simulink model "eml_hdl_design_patterns"  (R2026a)
settings: Solver=FixedStepDiscrete  StopTime=10
InitFcn:
  | errMsg  = ['\n\nThis model is only for demonstration purposes.\n\nPlease do not Simulate or code generate directly from this model. \n\nBefore generating code from this model please do copy the relevant blocks of interest from this model to a new model, place them in a subsystem, build a valid test bench around them.\n\nPlease refer to the example model ''eml_hdl_incrementer'' or HDLCoder documentation'];
  | error(sprintf(errMsg));
undefined symbols (not defined in the file or in its folder): C, gain_val, init_val, lower_limit, maxWordLength, thresh, upper_limit
libraries: simulink x2
(part 5 of 5)

== matlab function eml_hdl_design_patterns/Decoders/hierarchical_viterbi/PMU1/ACS ==
  settings: fimath=|
      | fimath(...
      |     'RoundMode', 'floor',...
      |     'OverflowMode', 'saturate',...
      |     'ProductMode', 'FullPrecision', 'ProductWordLength', 32,...
      |     'SumMode', 'FullPrecision', 'SumWordLength', 32,...
      |     'CastBeforeSum', true);
  data: nsm output; bm input; dec output; sm_reg input size=[1 64]
function [nsm,dec]  = ACSU(bm, sm_reg)
%--------------------------------------------------------------------------
%  ACS (Add-Compare-Select) block
%--------------------------------------------------------------------------

[nsm, dec] = acsunitbutterfly(bm, sm_reg);
   
end

%--------------------------------------------------------------------------
% ACS Unit Group(Add-Compare-Select)
% For each state in the trellis diagram, for each node in this state:
% 1. Add the branch metric to the paths merged to this node. 
% 2. Compare all the paths merged to this road
% 3. Select the path with the minimum path metric
%
% The following code is generated by a script 'generateviterbi.m'
% that generates trellis diagram for convolution code (7,171,133)
%--------------------------------------------------------------------------
function [nsm, dec] = acsunitbutterfly(bm, sm)

nsm = getfi(zeros(1,64),1, 12, 6);
dec = getfi(zeros(1,64),0, 1,  0);

%----------------------------------------------------
% 000000   -> 00 -> 000000   000001   -> 11 -> 000000   
%----------------------------------------------------
[nsm(1), dec(1)] = acsunit(bm(1),bm(4),sm(1),sm(2));
%----------------------------------------------------
% 000000   -> 11 -> 100000   000001   -> 00 -> 100000   
%----------------------------------------------------
[nsm(33), dec(33)] = acsunit(bm(4),bm(1),sm(1),sm(2));
%----------------------------------------------------
% 000010   -> 01 -> 000001   000011   -> 10 -> 000001   
%----------------------------------------------------
[nsm(2), dec(2)] = acsunit(bm(2),bm(3),sm(3),sm(4));
%----------------------------------------------------
% 000010   -> 10 -> 100001   000011   -> 01 -> 100001   
%----------------------------------------------------
[nsm(34), dec(34)] = acsunit(bm(3),bm(2),sm(3),sm(4));
%----------------------------------------------------
% 000100   -> 00 -> 000010   000101   -> 11 -> 000010   
%----------------------------------------------------
[nsm(3), dec(3)] = acsunit(bm(1),bm(4),sm(5),sm(6));
%----------------------------------------------------
% 000100   -> 11 -> 100010   000101   -> 00 -> 100010   
%----------------------------------------------------
[nsm(35), dec(35)] = acsunit(bm(4),bm(1),sm(5),sm(6));
%----------------------------------------------------
% 000110   -> 01 -> 000011   000111   -> 10 -> 000011   
%----------------------------------------------------
[nsm(4), dec(4)] = acsunit(bm(2),bm(3),sm(7),sm(8));
%----------------------------------------------------
% 000110   -> 10 -> 100011   000111   -> 01 -> 100011   
%----------------------------------------------------
[nsm(36), dec(36)] = acsunit(bm(3),bm(2),sm(7),sm(8));
%----------------------------------------------------
% 001000   -> 11 -> 000100   001001   -> 00 -> 000100   
%----------------------------------------------------
[nsm(5), dec(5)] = acsunit(bm(4),bm(1),sm(9),sm(10));
%----------------------------------------------------
% 001000   -> 00 -> 100100   001001   -> 11 -> 100100   
%----------------------------------------------------
[nsm(37), dec(37)] = acsunit(bm(1),bm(4),sm(9),sm(10));
%----------------------------------------------------
% 001010   -> 10 -> 000101   001011   -> 01 -> 000101   
%----------------------------------------------------
[nsm(6), dec(6)] = acsunit(bm(3),bm(2),sm(11),sm(12));
%----------------------------------------------------
% 001010   -> 01 -> 100101   001011   -> 10 -> 100101   
%----------------------------------------------------
[nsm(38), dec(38)] = acsunit(bm(2),bm(3),sm(11),sm(12));
%----------------------------------------------------
% 001100   -> 11 -> 000110   001101   -> 00 -> 000110   
%----------------------------------------------------
[nsm(7), dec(7)] = acsunit(bm(4),bm(1),sm(13),sm(14));
%----------------------------------------------------
% 001100   -> 00 -> 100110   001101   -> 11 -> 100110   
%----------------------------------------------------
[nsm(39), dec(39)] = acsunit(bm(1),bm(4),sm(13),sm(14));
%----------------------------------------------------
% 001110   -> 10 -> 000111   001111   -> 01 -> 000111   
%----------------------------------------------------
[nsm(8), dec(8)] = acsunit(bm(3),bm(2),sm(15),sm(16));
%----------------------------------------------------
% 001110   -> 01 -> 100111   001111   -> 10 -> 100111   
%----------------------------------------------------
[nsm(40), dec(40)] = acsunit(bm(2),bm(3),sm(15),sm(16));
%----------------------------------------------------
% 010000   -> 11 -> 001000   010001   -> 00 -> 001000   
%----------------------------------------------------
[nsm(9), dec(9)] = acsunit(bm(4),bm(1),sm(17),sm(18));
%----------------------------------------------------
% 010000   -> 00 -> 101000   010001   -> 11 -> 101000   
%----------------------------------------------------
[nsm(41), dec(41)] = acsunit(bm(1),bm(4),sm(17),sm(18));
%----------------------------------------------------
% 010010   -> 10 -> 001001   010011   -> 01 -> 001001   
%----------------------------------------------------
[nsm(10), dec(10)] = acsunit(bm(3),bm(2),sm(19),sm(20));
%----------------------------------------------------
% 010010   -> 01 -> 101001   010011   -> 10 -> 101001   
%----------------------------------------------------
[nsm(42), dec(42)] = acsunit(bm(2),bm(3),sm(19),sm(20));
%----------------------------------------------------
% 010100   -> 11 -> 001010   010101   -> 00 -> 001010   
%----------------------------------------------------
[nsm(11), dec(11)] = acsunit(bm(4),bm(1),sm(21),sm(22));
%----------------------------------------------------
% 010100   -> 00 -> 101010   010101   -> 11 -> 101010   
%----------------------------------------------------
[nsm(43), dec(43)] = acsunit(bm(1),bm(4),sm(21),sm(22));
%----------------------------------------------------
% 010110   -> 10 -> 001011   010111   -> 01 -> 001011   
%----------------------------------------------------
[nsm(12), dec(12)] = acsunit(bm(3),bm(2),sm(23),sm(24));
%----------------------------------------------------
% 010110   -> 01 -> 101011   010111   -> 10 -> 101011   
%----------------------------------------------------
[nsm(44), dec(44)] = acsunit(bm(2),bm(3),sm(23),sm(24));
%----------------------------------------------------
% 011000   -> 00 -> 001100   011001   -> 11 -> 001100   
%----------------------------------------------------
[nsm(13), dec(13)] = acsunit(bm(1),bm(4),sm(25),sm(26));
%----------------------------------------------------
% 011000   -> 11 -> 101100   011001   -> 00 -> 101100   
%----------------------------------------------------
[nsm(45), dec(45)] = acsunit(bm(4),bm(1),sm(25),sm(26));
%----------------------------------------------------
% 011010   -> 01 -> 001101   011011   -> 10 -> 001101   
%----------------------------------------------------
[nsm(14), dec(14)] = acsunit(bm(2),bm(3),sm(27),sm(28));
%----------------------------------------------------
% 011010   -> 10 -> 101101   011011   -> 01 -> 101101   
%----------------------------------------------------
[nsm(46), dec(46)] = acsunit(bm(3),bm(2),sm(27),sm(28));
%----------------------------------------------------
% 011100   -> 00 -> 001110   011101   -> 11 -> 001110   
%----------------------------------------------------
[nsm(15), dec(15)] = acsunit(bm(1),bm(4),sm(29),sm(30));
%----------------------------------------------------
% 011100   -> 11 -> 101110   011101   -> 00 -> 101110   
%----------------------------------------------------
[nsm(47), dec(47)] = acsunit(bm(4),bm(1),sm(29),sm(30));
%----------------------------------------------------
% 011110   -> 01 -> 001111   011111   -> 10 -> 001111   
%----------------------------------------------------
[nsm(16), dec(16)] = acsunit(bm(2),bm(3),sm(31),sm(32));
%----------------------------------------------------
% 011110   -> 10 -> 101111   011111   -> 01 -> 101111   
%----------------------------------------------------
[nsm(48), dec(48)] = acsunit(bm(3),bm(2),sm(31),sm(32));
%----------------------------------------------------
% 100000   -> 10 -> 010000   100001   -> 01 -> 010000   
%----------------------------------------------------
[nsm(17), dec(17)] = acsunit(bm(3),bm(2),sm(33),sm(34));
%----------------------------------------------------
% 100000   -> 01 -> 110000   100001   -> 10 -> 110000   
%----------------------------------------------------
[nsm(49), dec(49)] = acsunit(bm(2),bm(3),sm(33),sm(34));
%----------------------------------------------------
% 100010   -> 11 -> 010001   100011   -> 00 -> 010001   
%----------------------------------------------------
[nsm(18), dec(18)] = acsunit(bm(4),bm(1),sm(35),sm(36));
%----------------------------------------------------
% 100010   -> 00 -> 110001   100011   -> 11 -> 110001   
%----------------------------------------------------
[nsm(50), dec(50)] = acsunit(bm(1),bm(4),sm(35),sm(36));
%----------------------------------------------------
% 100100   -> 10 -> 010010   100101   -> 01 -> 010010   
%----------------------------------------------------
[nsm(19), dec(19)] = acsunit(bm(3),bm(2),sm(37),sm(38));
%----------------------------------------------------
% 100100   -> 01 -> 110010   100101   -> 10 -> 110010   
%----------------------------------------------------
[nsm(51), dec(51)] = acsunit(bm(2),bm(3),sm(37),sm(38));
%----------------------------------------------------
% 100110   -> 11 -> 010011   100111   -> 00 -> 010011   
%----------------------------------------------------
[nsm(20), dec(20)] = acsunit(bm(4),bm(1),sm(39),sm(40));
%----------------------------------------------------
% 100110   -> 00 -> 110011   100111   -> 11 -> 110011   
%----------------------------------------------------
[nsm(52), dec(52)] = acsunit(bm(1),bm(4),sm(39),sm(40));
%----------------------------------------------------
% 101000   -> 01 -> 010100   101001   -> 10 -> 010100   
%----------------------------------------------------
[nsm(21), dec(21)] = acsunit(bm(2),bm(3),sm(41),sm(42));
%----------------------------------------------------
% 101000   -> 10 -> 110100   101001   -> 01 -> 110100   
%----------------------------------------------------
[nsm(53), dec(53)] = acsunit(bm(3),bm(2),sm(41),sm(42));
%----------------------------------------------------
% 101010   -> 00 -> 010101   101011   -> 11 -> 010101   
%----------------------------------------------------
[nsm(22), dec(22)] = acsunit(bm(1),bm(4),sm(43),sm(44));
%----------------------------------------------------
% 101010   -> 11 -> 110101   101011   -> 00 -> 110101   
%----------------------------------------------------
[nsm(54), dec(54)] = acsunit(bm(4),bm(1),sm(43),sm(44));
%----------------------------------------------------
% 101100   -> 01 -> 010110   101101   -> 10 -> 010110   
%----------------------------------------------------
[nsm(23), dec(23)] = acsunit(bm(2),bm(3),sm(45),sm(46));
%----------------------------------------------------
% 101100   -> 10 -> 110110   101101   -> 01 -> 110110   
%----------------------------------------------------
[nsm(55), dec(55)] = acsunit(bm(3),bm(2),sm(45),sm(46));
%----------------------------------------------------
% 101110   -> 00 -> 010111   101111   -> 11 -> 010111   
%----------------------------------------------------
[nsm(24), dec(24)] = acsunit(bm(1),bm(4),sm(47),sm(48));
%----------------------------------------------------
% 101110   -> 11 -> 110111   101111   -> 00 -> 110111   
%----------------------------------------------------
[nsm(56), dec(56)] = acsunit(bm(4),bm(1),sm(47),sm(48));
%----------------------------------------------------
% 110000   -> 01 -> 011000   110001   -> 10 -> 011000   
%----------------------------------------------------
[nsm(25), dec(25)] = acsunit(bm(2),bm(3),sm(49),sm(50));
%----------------------------------------------------
% 110000   -> 10 -> 111000   110001   -> 01 -> 111000   
%----------------------------------------------------
[nsm(57), dec(57)] = acsunit(bm(3),bm(2),sm(49),sm(50));
%----------------------------------------------------
% 110010   -> 00 -> 011001   110011   -> 11 -> 011001   
%----------------------------------------------------
[nsm(26), dec(26)] = acsunit(bm(1),bm(4),sm(51),sm(52));
%----------------------------------------------------
% 110010   -> 11 -> 111001   110011   -> 00 -> 111001   
%----------------------------------------------------
[nsm(58), dec(58)] = acsunit(bm(4),bm(1),sm(51),sm(52));
%----------------------------------------------------
% 110100   -> 01 -> 011010   110101   -> 10 -> 011010   
%----------------------------------------------------
[nsm(27), dec(27)] = acsunit(bm(2),bm(3),sm(53),sm(54));
%----------------------------------------------------
% 110100   -> 10 -> 111010   110101   -> 01 -> 111010   
%----------------------------------------------------
[nsm(59), dec(59)] = acsunit(bm(3),bm(2),sm(53),sm(54));
%----------------------------------------------------
% 110110   -> 00 -> 011011   110111   -> 11 -> 011011   
%----------------------------------------------------
[nsm(28), dec(28)] = acsunit(bm(1),bm(4),sm(55),sm(56));
%----------------------------------------------------
% 110110   -> 11 -> 111011   110111   -> 00 -> 111011   
%----------------------------------------------------
[nsm(60), dec(60)] = acsunit(bm(4),bm(1),sm(55),sm(56));
%----------------------------------------------------
% 111000   -> 10 -> 011100   111001   -> 01 -> 011100   
%----------------------------------------------------
[nsm(29), dec(29)] = acsunit(bm(3),bm(2),sm(57),sm(58));
%----------------------------------------------------
% 111000   -> 01 -> 111100   111001   -> 10 -> 111100   
%----------------------------------------------------
[nsm(61), dec(61)] = acsunit(bm(2),bm(3),sm(57),sm(58));
%----------------------------------------------------
% 111010   -> 11 -> 011101   111011   -> 00 -> 011101   
%----------------------------------------------------
[nsm(30), dec(30)] = acsunit(bm(4),bm(1),sm(59),sm(60));
%----------------------------------------------------
% 111010   -> 00 -> 111101   111011   -> 11 -> 111101   
%----------------------------------------------------
[nsm(62), dec(62)] = acsunit(bm(1),bm(4),sm(59),sm(60));
%----------------------------------------------------
% 111100   -> 10 -> 011110   111101   -> 01 -> 011110   
%----------------------------------------------------
[nsm(31), dec(31)] = acsunit(bm(3),bm(2),sm(61),sm(62));
%----------------------------------------------------
% 111100   -> 01 -> 111110   111101   -> 10 -> 111110   
%----------------------------------------------------
[nsm(63), dec(63)] = acsunit(bm(2),bm(3),sm(61),sm(62));
%----------------------------------------------------
% 111110   -> 11 -> 011111   111111   -> 00 -> 011111   
%----------------------------------------------------
[nsm(32), dec(32)] = acsunit(bm(4),bm(1),sm(63),sm(64));
%----------------------------------------------------
% 111110   -> 00 -> 111111   111111   -> 11 -> 111111   
%----------------------------------------------------
[nsm(64), dec(64)] = acsunit(bm(1),bm(4),sm(63),sm(64));

end    
    
% ACS unit
function [select_metric, decision] = acsunit(branch_metric0, branch_metric1, stored_metric0, stored_metric1)

    % update branch0 metric
    a = getfi_sat(branch_metric0 + stored_metric0, 1, 12, 6);

    % update branch1 metric
    b = getfi_sat(branch_metric1 + stored_metric1, 1, 12, 6);
    
    % choose the metric
    if (a <= b)
        select_metric = a;
        decision = getfi(0, 0, 1, 0);
    else
        select_metric = b;
        decision = getfi(1, 0, 1, 0);
    end
end

function myfi = getfi(input, issigned, wlen, flen)

fm = fimath(...
    'RoundMode', 'floor',...
    'OverflowMode', 'wrap',...
    'ProductMode', 'FullPrecision', 'ProductWordLength', 32,...
    'SumMode', 'FullPrecision', 'SumWordLength', 32,...
    'CastBeforeSum', true);

myfi = fi(input, issigned, wlen, flen, 'fimath', fm);

end


function myfi = getfi_sat(input, issigned, wlen, flen)

fm_sat = fimath(...
    'RoundMode', 'floor',...
    'OverflowMode', 'saturate',...
    'ProductMode', 'FullPrecision', 'ProductWordLength', 32,...
    'SumMode', 'FullPrecision', 'SumWordLength', 32,...
    'CastBeforeSum', true);

myfi = fi(input, issigned, wlen, flen, 'fimath', fm_sat);

end

== matlab function eml_hdl_design_patterns/Decoders/hierarchical_viterbi/PMU1/ReNorm ==
  settings: fimath=|
      | fimath(...
      |     'RoundMode', 'floor',...
      |     'OverflowMode', 'saturate',...
      |     'ProductMode', 'FullPrecision', 'ProductWordLength', 32,...
      |     'SumMode', 'FullPrecision', 'SumWordLength', 32,...
      |     'CastBeforeSum', true);
  data: idx input; minimum input; nsm input; sm_next output; index output fixdt(0,8,0) size=1
function [sm_next, index]  = Renorm(idx, minimum, nsm)

%--------------------------------------------------------------------------
% Renormalize Block
% Finds the state with minimum path metric and outputs its index
% Then renormalizes all the path metrics by subsracting the minimum metric
%--------------------------------------------------------------------------
index = getfi((idx-1), 0, 8, 0);
sm_next = getfi_sat((nsm - minimum), 1, 12, 6);
    
end


function myfi = getfi(input, issigned, wlen, flen)

fm = fimath(...
    'RoundMode', 'floor',...
    'OverflowMode', 'wrap',...
    'ProductMode', 'FullPrecision', 'ProductWordLength', 32,...
    'SumMode', 'FullPrecision', 'SumWordLength', 32,...
    'CastBeforeSum', true);

myfi = fi(input, issigned, wlen, flen, 'fimath', fm);

end


function myfi = getfi_sat(input, issigned, wlen, flen)

fm_sat = fimath(...
    'RoundMode', 'floor',...
    'OverflowMode', 'saturate',...
    'ProductMode', 'FullPrecision', 'ProductWordLength', 32,...
    'SumMode', 'FullPrecision', 'SumWordLength', 32,...
    'CastBeforeSum', true);

myfi = fi(input, issigned, wlen, flen, 'fimath', fm_sat);

end

== matlab function eml_hdl_design_patterns/Decoders/hierarchical_viterbi/PMU1/TreeMin ==
  settings: fimath=|
      | fimath(...
      |     'RoundMode', 'floor',...
      |     'OverflowMode', 'wrap',...
      |     'ProductMode', 'FullPrecision', 'ProductWordLength', 32,...
      |     'SumMode', 'FullPrecision', 'SumWordLength', 32,...
      |     'CastBeforeSum', true);
  data: idx output; nsm input fixdt(1,12,6) size=[1 64]; minimum output
function [idx, minimum]  = TreeMin(nsm)
%--------------------------------------------------------------------------
% Tree implementation min function for vector input of length 64
%--------------------------------------------------------------------------
[minimum, idx] = tree_min(nsm);
            
end

function [minval, idx] = tree_min(invec)

% initialize outputs
% minval = getfi(0, 1, 12, 6);
% idx = 0;

% first level of comparison
inidx = uint8(1:64);
[lvlonemin, lvloneidx] = vector_min(invec, inidx);

% second level of comparison
[lvltwomin, lvltwoidx] = vector_min(lvlonemin, lvloneidx);

% third level of comparison
[lvlthreemin, lvlthreeidx] = vector_min(lvltwomin, lvltwoidx);

% fourth level of comparison
[lvlfourmin, lvlfouridx] = vector_min(lvlthreemin, lvlthreeidx);

% fifth level of comparison
[lvlfivemin, lvlfiveidx] = vector_min(lvlfourmin, lvlfouridx);

% final comparison
[minval, idx] = vector_min(lvlfivemin, lvlfiveidx);

end

% Minimum subfuction for tree implementation
function [minvec, idxvec] = vector_min(invec, inidx)
    
lengthminvec = uint8(length(invec)/2);
%lengthminvec = uint8(bitshift(invec, -1));
minvec = getfi(zeros(lengthminvec, 1), 1, 12, 6);
idxvec = uint8(zeros(lengthminvec, 1));

for i=1:lengthminvec
    % get two consecutive values
    idx2 = int8(i)+int8(i); %i*2
    idx1 = int8(idx2) - int8(1); %i*2-1
    % get elements
    val1 = invec(idx1);
    val2 = invec(idx2);
    % compare them and select minimum
    if le(val1, val2)
        minvec(i) = val1;
        idxvec(i) = inidx(idx1);
    else
        minvec(i) = val2;
        idxvec(i) = inidx(idx2);
    end
end

end


function myfi = getfi(input, issigned, wlen, flen)

fm = fimath(...
    'RoundMode', 'floor',...
    'OverflowMode', 'wrap',...
    'ProductMode', 'FullPrecision', 'ProductWordLength', 32,...
    'SumMode', 'FullPrecision', 'SumWordLength', 32,...
    'CastBeforeSum', true);

myfi = fi(input, issigned, wlen, flen, 'fimath', fm);

end

== matlab function eml_hdl_design_patterns/Decoders/hierarchical_viterbi/TBU1 ==
  settings: fimath=|
      | fimath(...
      | 'RoundMode', 'floor',...
      | 'OverflowMode', 'wrap',...
      | 'ProductMode', 'FullPrecision', 'ProductWordLength', 32,...
      | 'SumMode', 'FullPrecision', 'SumWordLength', 32,...
      | 'CastBeforeSum', true)
  data: dec input; index input fixdt(0,8,0) size=1; y output
function y = TBU(dec, index)

% traceback storage register
persistent tb_reg;  
if isempty(tb_reg)
    tb_reg = getfi(zeros(1,64), 0, 27, 0);
end

% traceback output register
persistent tbout_reg
if isempty(tbout_reg)
    tbout_reg = getfi(0,0,1,0);
end
    
%--------------------------------------------------------------------------
% TBU (Trace Back Unit)
% Trace back unit restore the optimal path information stored in the 
% path metric register. The trace back depth of this decoder is 32 steps,
% which means every decoded symbol is based on the minimum path metric in the
% following 32 steps. 
%
% The trace back unit is implemented by a 27 stage shift register.
% Only 27 stage is necessary (instead of 32) because we can retrieve the 
% input symbol of the 32th stage from the shift register index of the 27th stage.
%
% Normal implementation uses 27 64-bit registers for trance back unit. 
% We use 64 27-bit registers instead because of the fixed-point bitwidth limit.
%--------------------------------------------------------------------------

% stores path metric decision inforamtion from PMU unit
tb_reg = bitshift(tb_reg, 1);
tb_reg = bitset(tb_reg, ones(1,64), uint8(dec));

% trace back unit
for i=1:27
  index = tbunit(index, tb_reg, i);
end

% the LSB of the 27th trace back step is the decoder output
tbmask = getfi(1, 0, 8, 0);
tband = bitand(index, tbmask);

% register the final result
prev_result = tbout_reg;
tbout_reg = getfi(tband, 0, 1, 0);

% update output as boolean datatype
y =  (prev_result == getfi(1, 0, 1, 0));

end

%--------------------------------------------------------------------------
% TB Unit (Trace Back Unit)
% Given the index of the minimum metric node in the current stages,
% also given the stored decision information in the current stages,
% we can restore the index of the minimum metric node in the previous stage.
%--------------------------------------------------------------------------
function new_idx = tbunit (current_idx, tb_reg, stage)

idx = int8(current_idx) + int8(1);
tbread = bitget(tb_reg(idx), stage);

tbshift = bitshift(current_idx, 1);
tband = bitand(tbshift, getfi(62, 0, 8, 0));
new_idx = bitor(tband, getfi(tbread, 0, 8, 0));

end


function myfi = getfi(input, issigned, wlen, flen)

fm = fimath(...
    'RoundMode', 'floor',...
    'OverflowMode', 'wrap',...
    'ProductMode', 'FullPrecision', 'ProductWordLength', 32,...
    'SumMode', 'FullPrecision', 'SumWordLength', 32,...
    'CastBeforeSum', true);

myfi = fi(input, issigned, wlen, flen, 'fimath', fm);

end

== matlab function eml_hdl_design_patterns/Complex/Complex Transpose ==
  settings: fimath=|
      | fimath(...
      | 'RoundMode', 'floor',...
      | 'OverflowMode', 'wrap',...
      | 'ProductMode', 'FullPrecision', 'ProductWordLength', 32,...
      | 'SumMode', 'FullPrecision', 'SumWordLength', 32,...
      | 'CastBeforeSum', true)
  data: ct output; c input
function ct = fcn(c)
% Compute Complex (non-conjugate) transpose of c

ct = c.';

== matlab function eml_hdl_design_patterns/Counters/counter_clear ==
  settings: fimath=|
      | fimath(...
      | 'RoundMode', 'floor',...
      | 'OverflowMode', 'wrap',...
      | 'ProductMode', 'FullPrecision', 'ProductWordLength', 32,...
      | 'SumMode', 'FullPrecision', 'SumWordLength', 32,...
      | 'CastBeforeSum', true)
  data: clear input boolean; count output fixdt(0,4,0) size=1
function count  = fcn(clear)

% A counter with synchronous clear, that counts how many times
% this block is called.
% 'count' saturates if called more than 15 times.
% Set 'OverflowMode' of result_fm to 'wrap' if you want the counter
% to roll over.

result_nt = numerictype(0,4,0);
result_fm = fimath('OverflowMode', 'saturate', 'RoundMode', 'floor');

persistent count_reg;
if isempty(count_reg)
    count_reg = fi(0, result_nt, result_fm);
end

count = count_reg;

if clear
    count_reg = fi(0, result_nt, result_fm);
else    
    inc = count_reg + fi(1, result_nt, result_fm);
    count_reg = fi(inc, result_nt, result_fm);
end

== matlab function eml_hdl_design_patterns/Complex/Complex Conj Transpose ==
  settings: fimath=|
      | fimath(...
      | 'RoundMode', 'floor',...
      | 'OverflowMode', 'wrap',...
      | 'ProductMode', 'FullPrecision', 'ProductWordLength', 32,...
      | 'SumMode', 'FullPrecision', 'SumWordLength', 32,...
      | 'CastBeforeSum', true)
  data: ct output; c input
function ct = fcn(c)
% Compute Complex conjugate transpose of c

ct = c';

== matlab function eml_hdl_design_patterns/Complex/Complex Constant ==
  settings: fimath=|
      | fimath(...
      | 'RoundMode', 'floor',...
      | 'OverflowMode', 'wrap',...
      | 'ProductMode', 'FullPrecision', 'ProductWordLength', 32,...
      | 'SumMode', 'FullPrecision', 'SumWordLength', 32,...
      | 'CastBeforeSum', true)
  data: sc output; vc output
function [sc, vc] = fcn
% Compute Constant

f = fimath;
nt = numerictype(0, 16, 2);

% scalar constant
sc = fi(complex(-1), nt, f);

% vector constant
vc = fi(complex(zeros(1,4)), nt, f);

== matlab function eml_hdl_design_patterns/Complex/Complex Add ==
  settings: fimath=|
      | fimath(...
      | 'RoundMode', 'floor',...
      | 'OverflowMode', 'wrap',...
      | 'ProductMode', 'FullPrecision', 'ProductWordLength', 32,...
      | 'SumMode', 'FullPrecision', 'SumWordLength', 32,...
      | 'CastBeforeSum', true)
  data: out output; in1 input fixdt(1,14,2); in2 input fixdt(1,14,2)
function out = fcn(in1, in2)
% Compute Addition
%
%  out_re = in1_re + in2_re
%  out_im = in1_im + in2_im
%
% For fixed point inputs 'SumMode' option on the block fimath 
% decides the sum semantic. In this example SumMode is set to FullPrecision 
% which is optimal for HDLCodegen


f = fimath(in1);
nt = numerictype(in1);

out = fi(in1 + in2, nt, f);

== matlab function eml_hdl_design_patterns/Complex/Complex Sub ==
  settings: fimath=|
      | fimath(...
      | 'RoundMode', 'floor',...
      | 'OverflowMode', 'wrap',...
      | 'ProductMode', 'FullPrecision', 'ProductWordLength', 32,...
      | 'SumMode', 'FullPrecision', 'SumWordLength', 32,...
      | 'CastBeforeSum', true)
  data: out output; in1 input fixdt(1,14,2); in2 input fixdt(1,14,2)
function out = fcn(in1, in2)
% Compute Subtraction
%
%  out_re = in1_re - in2_re
%  out_im = in1_im - in2_im
%
% For fixed point inputs 'SumMode' option on the block fimath 
% decides the sum semantic. In this example SumMode is set to FullPrecision 
% which is optimal for HDLCodegen


f = fimath(in1);
nt = numerictype(in1);

out = fi(in1 - in2, nt, f);

== matlab function eml_hdl_design_patterns/Delays/Unit Delay ==
  settings: fimath=|
      | fimath(...
      | 'RoundMode', 'floor',...
      | 'OverflowMode', 'wrap',...
      | 'ProductMode', 'FullPrecision', 'ProductWordLength', 32,...
      | 'SumMode', 'FullPrecision', 'SumWordLength', 32,...
      | 'CastBeforeSum', true)
  data: u input; y output
function y = fcn(u)
% Complex unit delay

% The Unit Delay block delays its input by the specified sample period.
% The block accepts one input and generates one output, which can
% be either both scalar or both vector. If the input is a vector, 
% all elements of the vector are delayed by the same sample period.
%
% You specify the block output for the first sampling period with the 
% Initial value to the persistent variable.
%

% y is same as u delayed by one sample period.

% output of this block at the first sample hit is decided by the initial 
% value of this persistent variable.

persistent u_d;
if isempty(u_d)
    % defines initial value driven by unit delay at time step 0
    u_d = fi(0, numerictype(u), fimath(u));
end

% return delayed input from last sample time hit
y = u_d;

% store the current input to be used later
u_d = u;

== matlab function eml_hdl_design_patterns/Complex/Complex Switch ==
  settings: fimath=|
      | fimath(...
      | 'RoundMode', 'floor',...
      | 'OverflowMode', 'wrap',...
      | 'ProductMode', 'FullPrecision', 'ProductWordLength', 32,...
      | 'SumMode', 'FullPrecision', 'SumWordLength', 32,...
      | 'CastBeforeSum', true)
  data: out output; in1 input; in2 input; ctrl input boolean
function out = fcn(in1, in2, ctrl)
% Complex switch

if (ctrl)
    out = in1;
else
    out = in2;
end
